simulink model "W10A_LoopShaping"  (R2024b)
settings: Solver=ode45  StartTime=0.0  StopTime=t_end  MaxStep=2e-4  RelTol=1e-3
PreLoadFcn:
  | % W10A_LoopShaping 기본 파라미터 (모델을 열 때 자동 실행)
  | % 플랜트 P = 0.1/(0.5s+2),  제어기 C = (500s+2000)/s  ->  L = 100/s
  | defs = { 'r_amp',1 ;
  |          'numC',[500 2000] ; 'denC',[1 0] ;
  |          'numP',0.1        ; 'denP',[0.5 2] ;
  |          'd_amp',0.3       ; 'w_d',2*pi ;
  |          'noise_pow',2e-7  ; 'noise_ts',5e-4 ;
  |          't_end',2 };
  | for ii = 1:size(defs,1)
  |     if ~evalin('base', sprintf('exist(''%s'',''var'')', defs{ii,1}))
  |         assignin('base', defs{ii,1}, defs{ii,2});
  |     end
  | end
  | clear defs ii
values from neighbouring files (symbols this model uses):
  d_amp = 0    [W10A_05_run_simulink.m]
  denC = [1 0]    [W10A_05_run_simulink.m]
  denP = [0.5 2]    [W10A_05_run_simulink.m]
  noise_ts = 1e-4    (= 0.0001)    [W10A_04_disturbance_noise.m]    (also in W10A_05_run_simulink.m = 0.0005)
  numC = [500 2000]    [W10A_05_run_simulink.m]
  numP = 0.1    [W10A_05_run_simulink.m]
  r_amp = 0    [W10A_05_run_simulink.m]
  w_d = 2*pi    (= 6.28318530718)    [W10A_05_run_simulink.m]
libraries: simulink x1
settings Model: Creator=admin  LastModifiedBy=admin

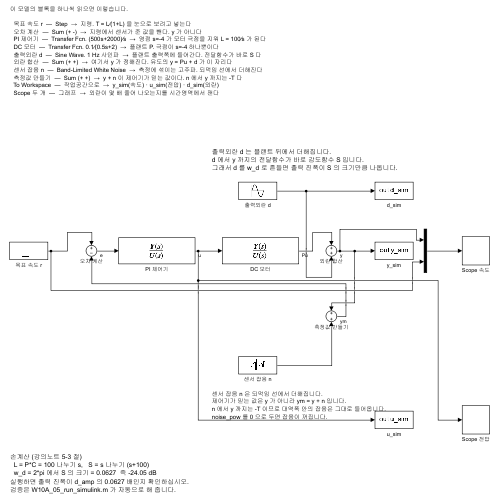
[thumbnail: Simulink's stored preview of the top-level diagram]
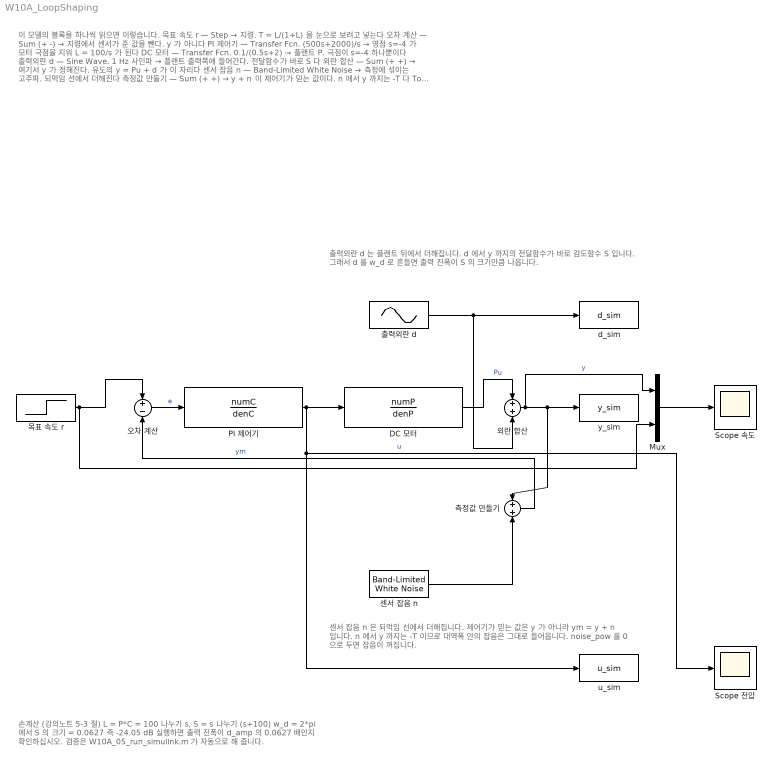
== system W10A_LoopShaping ==
  note: 출력외란 d 는 플랜트 뒤에서 더해집니다.
      | d 에서 y 까지의 전달함수가 바로 감도함수 S 입니다.
      | 그래서 d 를 w_d 로 흔들면 출력 진폭이 S 의 크기만큼 나옵니다.
  note: 센서 잡음 n 은 되먹임 선에서 더해집니다.
      | 제어기가 믿는 값은 y 가 아니라 ym = y + n 입니다.
      | n 에서 y 까지는 -T 이므로 대역폭 안의 잡음은 그대로 들어옵니다.
      | noise_pow 를 0 으로 두면 잡음이 꺼집니다.
  note: 손계산 (강의노트 5-3 절)
      |   L = P*C = 100 나누기 s,   S = s 나누기 (s+100)
      |   w_d = 2*pi 에서 S 의 크기 = 0.0627  즉 -24.05 dB
      | 실행하면 출력 진폭이 d_amp 의 0.0627 배인지 확인하십시오.
      | 검증은 W10A_05_run_simulink.m 가 자동으로 해 줍니다.
  note: 이 모델의 블록을 하나씩 읽으면 이렇습니다.
      |
      |   목표 속도 r  —  Step  →  지령. T = L∕(1+L) 을 눈으로 보려고 넣는다
      |   오차 계산  —  Sum (+ -)  →  지령에서 센서가 준 값을 뺀다. y 가 아니다
      |   PI 제어기  —  Transfer Fcn. (500s+2000)∕s  →  영점 s=-4 가 모터 극점을 지워 L = 100∕s 가 된다
      |   DC 모터  —  Transfer Fcn. 0.1∕(0.5s+2)  →  플랜트 P. 극점이 s=-4 하나뿐이다
      |   출력외란 d  —  Sine Wave. 1 Hz 사인파  →  플랜트 출력쪽에 들어간다. 전달함수가 바로 S 다
      |   외란 합산  —  Sum (+ +)  →  여기서 y 가 정해진다. 유도의 y = Pu + d 가 이 자리다
      |   센서 잡음 n  —  Band-Limited White Noise  →  측정에 섞이는 고주파. 되먹임 선에서 더해진다
      |   측정값 만들기  —  Sum (+ +)  →  y + n 이 제어기가 믿는 값이다. n 에서 y 까지는 -T 다
      |   To Workspace  —  작업공간으로  →  y_sim(속도) · u_sim(전압) · d_sim(외란)
      |   Scope 두 개  —  그래프  →  외란이 몇 배 줄어 나오는지를 시간영역에서 잰다
  DC 모터 : TransferFcn  Numerator=numP  Denominator=denP
  Mux : Mux  Inputs=2
  PI 제어기 : TransferFcn  Numerator=numC  Denominator=denC
  Scope 속도 : Scope
  Scope 전압 : Scope
  d_sim : ToWorkspace  VariableName=d_sim  SaveFormat=Timeseries  SampleTime=-1
  u_sim : ToWorkspace  VariableName=u_sim  SaveFormat=Timeseries  SampleTime=-1
  y_sim : ToWorkspace  VariableName=y_sim  SaveFormat=Timeseries  SampleTime=-1
  목표 속도 r : Step  Time=0  After=r_amp  SampleTime=0
  센서 잡음 n : simulink/Sources/Band-Limited White Noise  Cov=noise_pow  Ts=noise_ts  seed=12345
  오차 계산 : Sum  Inputs=+-
  외란 합산 : Sum
  출력외란 d : Sin  Amplitude=d_amp  Frequency=w_d  SampleTime=0
  측정값 만들기 : Sum
  wires:
  목표 속도 r/1 -> 오차 계산/1, Mux/2
  오차 계산/1 -> PI 제어기/1  "e"
  PI 제어기/1 -> u_sim/1, Scope 전압/1, DC 모터/1  "u"
  DC 모터/1 -> 외란 합산/1  "Pu"
  출력외란 d/1 -> 외란 합산/2, d_sim/1
  외란 합산/1 -> y_sim/1, 측정값 만들기/1, Mux/1  "y"
  Mux/1 -> Scope 속도/1
  센서 잡음 n/1 -> 측정값 만들기/2
  측정값 만들기/1 -> 오차 계산/2  "ym"
